simulink model "ranwalk_kalman"  (Simulink 5.0)
settings: Solver=ode45  StartTime=0.0  StopTime=100.0  RelTol=1e-3
values from neighbouring files (symbols this model uses):
  H = [1 0 1 1 1 1 1 1 1 1 1 1 ... (56 elements, 2x28)]    [cmigits28_model_01.mat]    (also in covanal.m = zeros(1,28))
  P0 = covupdate(P1,K,H)    [casimple.m]    (also in cmigits28_model_01.mat = [100 0 0 0 0 0 0 0 0 0 0 0 ... (784 elements, 28x28)])
  Phi = expm(F)    [casimple.m]    (also in covanal.m = eye(28))
  Q = [100 0 0 0 0 0 0 0 0 0 0 0 ... (784 elements, 28x28)]    [cmigits28_model_01.mat]    (also in covanal.m = eye(28))
  R = Re + h    (= 6378441.8)    [A-init.m]    (also in Ainit.m; cmigits28_model_01.mat = [50  0; 0  50]; covanal.m = zeros(1,1); covariance_analysis.m = meas_noise_growth_factor*R)
  x0 = [lat,lon,Vn,Ve,0,0,0,-R,0]'    [Ainit.m]
undefined symbols (not defined in the file or in its folder): rss_ratio, trace, ud_inv
libraries: simulink x4
settings Model: Creator=mcarroll  LastModifiedBy=mcarroll  ExtModeAutoUpdateStatusClock=off  SaveFormat=StructureWithTime

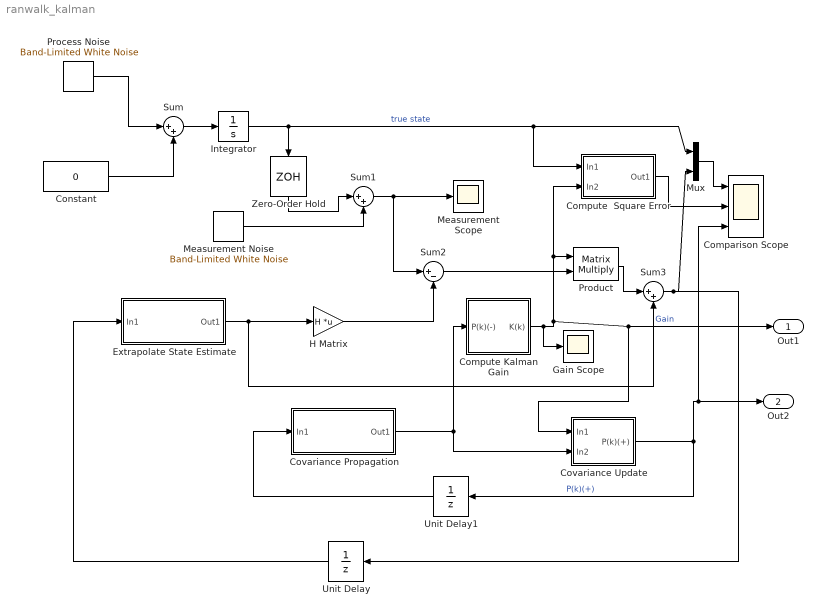
== system ranwalk_kalman ==
  Comparison Scope : Scope  NumInputPorts=3
      settings: TimeRange=100  YMin=1.5~-5~-5  YMax=6.5~5~5  SaveName=ScopeData12
  Compute Kalman Gain : Subsystem
  Compute  Square Error : Subsystem
  Constant : Constant  Value=0
  Covariance Propagation : Subsystem
  Covariance Update : Subsystem
  Extrapolate State Estimate : Subsystem
  Gain Scope : Scope
  H Matrix : Gain  Gain=H  Multiplication=Matrix(K*u)  SaturateOnIntegerOverflow=on
  Integrator : Integrator  InitialCondition=5+randn
  Measurement Noise : simulink/Sources/Band-Limited White Noise  Cov=[0.01]  Ts=0.1  seed=[23341]
  Measurement Scope : Scope
  Mux : Mux  Inputs=2
  Process Noise : simulink/Sources/Band-Limited White Noise  Cov=[10]  Ts=0.1  seed=[23341]
  Product : Product  Multiplication=Matrix(*)  SaturateOnIntegerOverflow=on
  Sum : Sum  Inputs=|++  SaturateOnIntegerOverflow=on
  Sum1 : Sum  Inputs=|++  SaturateOnIntegerOverflow=on
  Sum2 : Sum  Inputs=|+-  SaturateOnIntegerOverflow=on
  Sum3 : Sum  Inputs=|++  SaturateOnIntegerOverflow=on
  Unit Delay : UnitDelay  Orientation=left  X0=x0
  Unit Delay1 : UnitDelay  Orientation=left  X0=P0
  Zero-Order Hold : ZeroOrderHold  Orientation=down
  Out1 : Outport
  Out2 : Outport  Port=2
  wires:
  Sum/1 -> Integrator/1
  Process Noise/1 -> Sum/1
  Constant/1 -> Sum/2
  Integrator/1 -> Zero-Order Hold/1, Mux/1, Compute  Square Error/1(In1)  "true state"
  Measurement Noise/1 -> Sum1/2
  Sum1/1 -> Measurement Scope/1, Sum2/1
  Extrapolate State Estimate/1(Out1) -> H Matrix/1, Sum3/2
  H Matrix/1 -> Sum2/2
  Sum3/1 -> Unit Delay/1, Mux/2
  Unit Delay/1 -> Extrapolate State Estimate/1(In1)
  Zero-Order Hold/1 -> Sum1/1
  Unit Delay1/1 -> Covariance Propagation/1(In1)
  Covariance Propagation/1(Out1) -> Compute Kalman Gain/1(P(k)(-)), Covariance Update/2(In2)
  Compute Kalman Gain/1(K(k)) -> Covariance Update/1(In1), Out1/1, Product/1, Compute  Square Error/2(In2), Gain Scope/1  "Gain"
  Covariance Update/1(P(k)(+)) -> Unit Delay1/1, Out2/1, Comparison Scope/3  "P(k)(+)"
  Product/1 -> Sum3/1
  Sum2/1 -> Product/2
  Mux/1 -> Comparison Scope/1
  Compute  Square Error/1(Out1) -> Comparison Scope/2

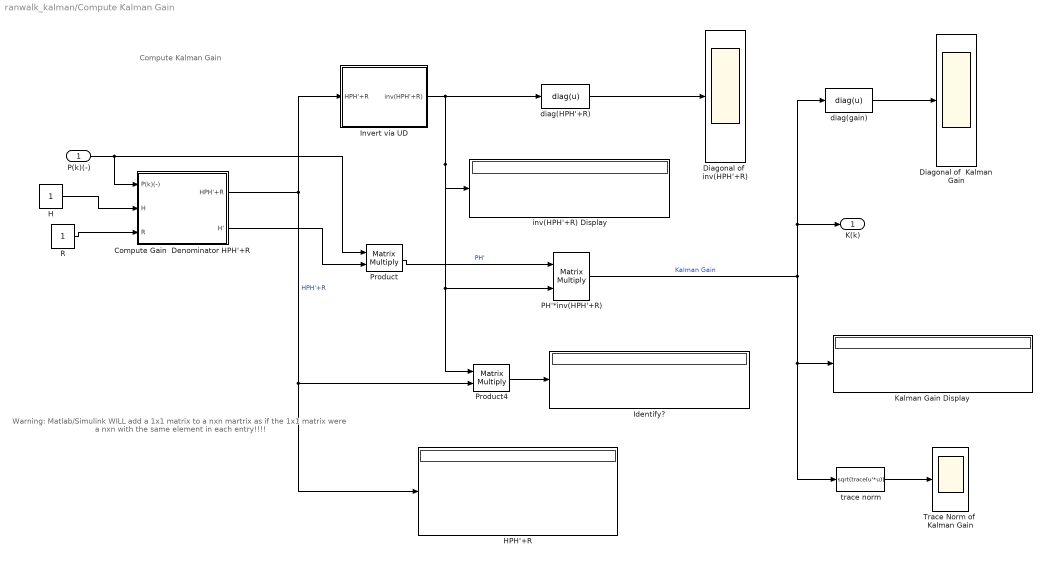
== system ranwalk_kalman/Compute Kalman Gain ==
  note: Compute Kalman Gain
  note: Warning:
      | Matlab/Simulink
      | WILL add a 1x1 matrix to
      | a nxn martrix as if the
      | 1x1 matrix were a
      | nxn with the same element
      | in each entry!!!!
  P(k)(-) : Inport  ShowAdditionalParam=on
  Compute Gain  Denominator HPH'+R : Subsystem
  Diagonal of  Kalman Gain : Scope
      settings: TimeRange=10  YMin=0  YMax=0.8  SaveName=ScopeData7
  Diagonal of  inv(HPH'+R) : Scope
      settings: TimeRange=100  YMin=0.0006  YMax=0.002  SaveName=ScopeData8
  H : Constant
  HPH'+R : Display
  Identify? : Display
  Invert via UD : Subsystem
  Kalman Gain Display : Display
  PH'*inv(HPH'+R) : Product  Multiplication=Matrix(*)  SaturateOnIntegerOverflow=on  InputSameDT=on
  Product : Product  Multiplication=Matrix(*)  SaturateOnIntegerOverflow=on
  Product4 : Product  Multiplication=Matrix(*)  SaturateOnIntegerOverflow=on  InputSameDT=on
  R : Constant
  Trace Norm of  Kalman Gain : Scope
      settings: TimeRange=10  YMin=0.5  YMax=0.62  SaveName=ScopeData11
  diag(HPH'+R) : MATLABFcn  MATLABFcn=diag(u)
  diag(gain) : MATLABFcn  MATLABFcn=diag(u)  Output1D=off
  inv(HPH'+R) Display : Display
  trace norm : MATLABFcn  MATLABFcn=sqrt(trace(u'*u))  Output1D=off
  K(k) : Outport
  wires:
  Compute Gain  Denominator HPH'+R/1(HPH'+R) -> Invert via UD/1(HPH'+R), HPH'+R/1, Product4/2  "HPH'+R"
  R/1 -> Compute Gain  Denominator HPH'+R/3(R)
  diag(HPH'+R)/1 -> Diagonal of  inv(HPH'+R)/1
  Invert via UD/1(inv(HPH'+R)) -> diag(HPH'+R)/1, inv(HPH'+R) Display/1, PH'*inv(HPH'+R)/2, Product4/1
  Compute Gain  Denominator HPH'+R/2(H') -> Product/2
  Product/1 -> PH'*inv(HPH'+R)/1  "PH'"
  diag(gain)/1 -> Diagonal of  Kalman Gain/1
  trace norm/1 -> Trace Norm of  Kalman Gain/1
  Product4/1 -> Identify?/1
  H/1 -> Compute Gain  Denominator HPH'+R/2(H)
  P(k)(-)/1 -> Compute Gain  Denominator HPH'+R/1(P(k)(-)), Product/1
  PH'*inv(HPH'+R)/1 -> K(k)/1, diag(gain)/1, Kalman Gain Display/1, trace norm/1  "Kalman Gain"

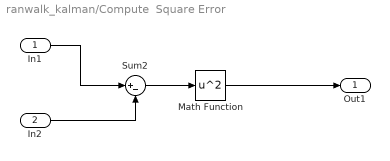
== system ranwalk_kalman/Compute  Square Error ==
  In1 : Inport
  In2 : Inport  Port=2
  Math Function : Math  Operator=square
  Sum2 : Sum  Inputs=|+-  SaturateOnIntegerOverflow=on
  Out1 : Outport
  wires:
  In1/1 -> Sum2/1
  In2/1 -> Sum2/2
  Sum2/1 -> Math Function/1
  Math Function/1 -> Out1/1

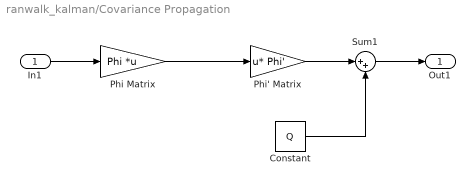
== system ranwalk_kalman/Covariance Propagation ==
  In1 : Inport
  Constant : Constant  Value=Q
  Phi Matrix : Gain  Gain=Phi  Multiplication=Matrix(K*u)  SaturateOnIntegerOverflow=on
  Phi' Matrix : Gain  Gain=Phi'  Multiplication=Matrix(u*K)  SaturateOnIntegerOverflow=on
  Sum1 : Sum  Inputs=|++  SaturateOnIntegerOverflow=on
  Out1 : Outport
  wires:
  In1/1 -> Phi Matrix/1
  Phi Matrix/1 -> Phi' Matrix/1
  Phi' Matrix/1 -> Sum1/1
  Constant/1 -> Sum1/2
  Sum1/1 -> Out1/1

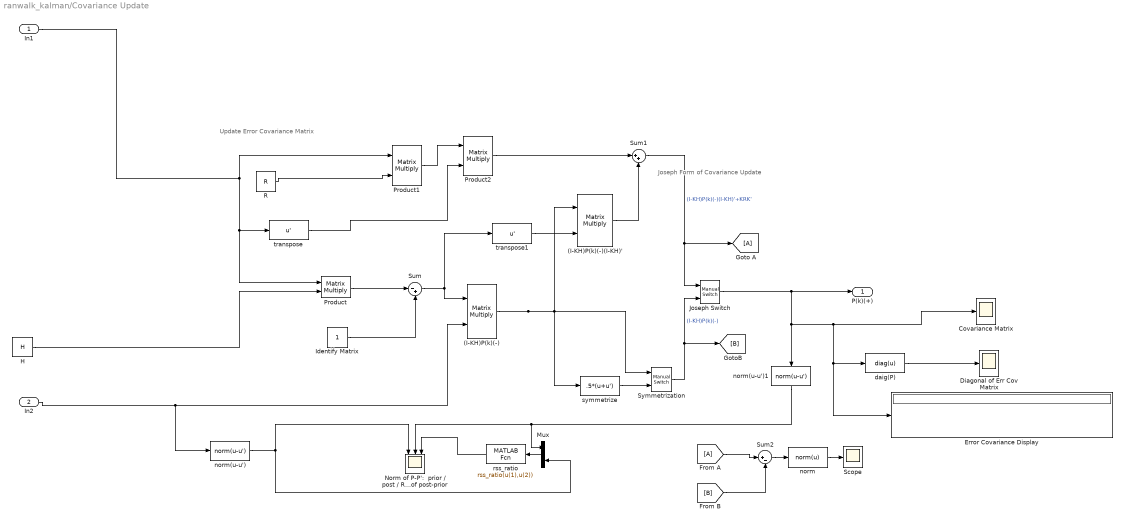
== system ranwalk_kalman/Covariance Update ==
  note: Update Error Covariance Matrix
  note: Joseph Form
      | of Covariance
      | Update
  In1 : Inport
  In2 : Inport  Port=2
  (I-KH)P(k)(-) : Product  Multiplication=Matrix(*)  SaturateOnIntegerOverflow=on  InputSameDT=on
  (I-KH)P(k)(-)(I-KH)' : Product  Multiplication=Matrix(*)  SaturateOnIntegerOverflow=on  InputSameDT=on
  Covariance Matrix : Scope
      settings: TimeRange=10  YMin=-60  YMax=80  SaveName=ScopeData2
  Diagonal of Err Cov Matrix : Scope
      settings: YMin=0  YMax=5000  SaveName=ScopeData3
  Error Covariance Display : Display
  H : Constant  Value=H  VectorParams1D=off
  Identify Matrix : Constant  VectorParams1D=off
  Joseph Switch : simulink/Signal Routing/Manual Switch  sw=1  action=0
  Mux : Mux  Orientation=left  Inputs=2
  Norm of P-P':  prior / post / RSS ratio of post-prior : Scope  NumInputPorts=3
      settings: Orientation=down  TimeRange=10  YMin=0~0~0  YMax=40~2~0.05  SaveName=ScopeData4
  Product : Product  Multiplication=Matrix(*)  SaturateOnIntegerOverflow=on  InputSameDT=on
  Product1 : Product  Multiplication=Matrix(*)  SaturateOnIntegerOverflow=on  InputSameDT=on
  Product2 : Product  Multiplication=Matrix(*)  ShowAdditionalParam=on  SaturateOnIntegerOverflow=on  InputSameDT=on
  R : Constant  Value=R  VectorParams1D=off
  Scope : Scope
      settings: SaveName=ScopeData5
  Sum : Sum  Inputs=|-+  SaturateOnIntegerOverflow=on  InputSameDT=on
  Sum1 : Sum  Inputs=|++  SaturateOnIntegerOverflow=on  InputSameDT=on
  Sum2 : Sum  Inputs=|+-  SaturateOnIntegerOverflow=on  InputSameDT=on
  Symmetrization : simulink/Signal Routing/Manual Switch  sw=1  action=0
  daig(P) : MATLABFcn  MATLABFcn=diag(u)
  norm : MATLABFcn  MATLABFcn=norm(u)  Output1D=off
  norm(u-u') : MATLABFcn  MATLABFcn=norm(u-u')  Output1D=off
  norm(u-u')1 : MATLABFcn  Orientation=down  MATLABFcn=norm(u-u')  Output1D=off
  rss_ratio : MATLABFcn  Orientation=left  MATLABFcn=rss_ratio(u(1),u(2))  OutputSignalType=real
  symmetrize : MATLABFcn  MATLABFcn=.5*(u+u')  Output1D=off
  transpose : MATLABFcn  MATLABFcn=u'  Output1D=off
  transpose1 : MATLABFcn  MATLABFcn=u'  Output1D=off
  P(k)(+) : Outport
  wires:
  H/1 -> Product/2
  In1/1 -> Product/1, transpose/1, Product1/1
  In2/1 -> (I-KH)P(k)(-)/2, norm(u-u')/1
  Identify Matrix/1 -> Sum/2
  Product/1 -> Sum/1
  Sum/1 -> (I-KH)P(k)(-)/1, transpose1/1
  R/1 -> Product1/2
  transpose/1 -> Product2/2
  (I-KH)P(k)(-)/1 -> (I-KH)P(k)(-)(I-KH)'/1, Symmetrization/1, symmetrize/1
  transpose1/1 -> (I-KH)P(k)(-)(I-KH)'/2
  (I-KH)P(k)(-)(I-KH)'/1 -> Sum1/2
  Product2/1 -> Sum1/1
  symmetrize/1 -> Symmetrization/2
  Symmetrization/1 -> Joseph Switch/2, [B]  "(I-KH)P(k)(-)"
  Joseph Switch/1 -> P(k)(+)/1, norm(u-u')1/1, daig(P)/1, Error Covariance Display/1, Covariance Matrix/1
  Sum1/1 -> Joseph Switch/1, [A]  "(I-KH)P(k)(-)(I-KH)'+KRK'"
  norm(u-u')/1 -> Norm of P-P':  prior / post / RSS ratio of post-prior/1, Mux/2
  norm(u-u')1/1 -> Norm of P-P':  prior / post / RSS ratio of post-prior/2, Mux/1
  rss_ratio/1 -> Norm of P-P':  prior / post / RSS ratio of post-prior/3
  Mux/1 -> rss_ratio/1
  [B] -> Sum2/2
  [A] -> Sum2/1
  Sum2/1 -> norm/1
  norm/1 -> Scope/1
  daig(P)/1 -> Diagonal of Err Cov Matrix/1
  Product1/1 -> Product2/1

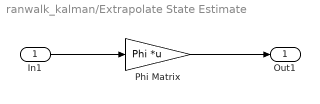
== system ranwalk_kalman/Extrapolate State Estimate ==
  In1 : Inport
  Phi Matrix : Gain  Gain=Phi  Multiplication=Matrix(K*u)  SaturateOnIntegerOverflow=on
  Out1 : Outport
  wires:
  In1/1 -> Phi Matrix/1
  Phi Matrix/1 -> Out1/1

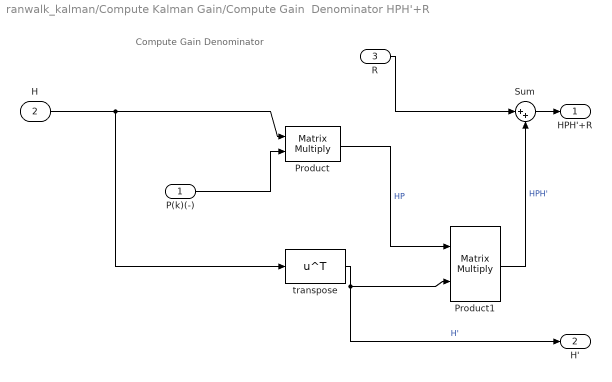
== system ranwalk_kalman/Compute Kalman Gain/Compute Gain  Denominator HPH'+R ==
  note: Compute Gain Denominator
  P(k)(-) : Inport
  H : Inport  Port=2
  R : Inport  Port=3
  Product : Product  Multiplication=Matrix(*)  SaturateOnIntegerOverflow=on  InputSameDT=on
  Product1 : Product  Multiplication=Matrix(*)  SaturateOnIntegerOverflow=on  InputSameDT=on
  Sum : Sum  Inputs=|++  SaturateOnIntegerOverflow=on  InputSameDT=on
  transpose : Math  Operator=transpose
  HPH'+R : Outport
  H' : Outport  Port=2
  wires:
  transpose/1 -> H'/1, Product1/2  "H'"
  Product1/1 -> Sum/2  "HPH'"
  Product/1 -> Product1/1  "HP"
  H/1 -> Product/1, transpose/1
  R/1 -> Sum/1
  Sum/1 -> HPH'+R/1
  P(k)(-)/1 -> Product/2

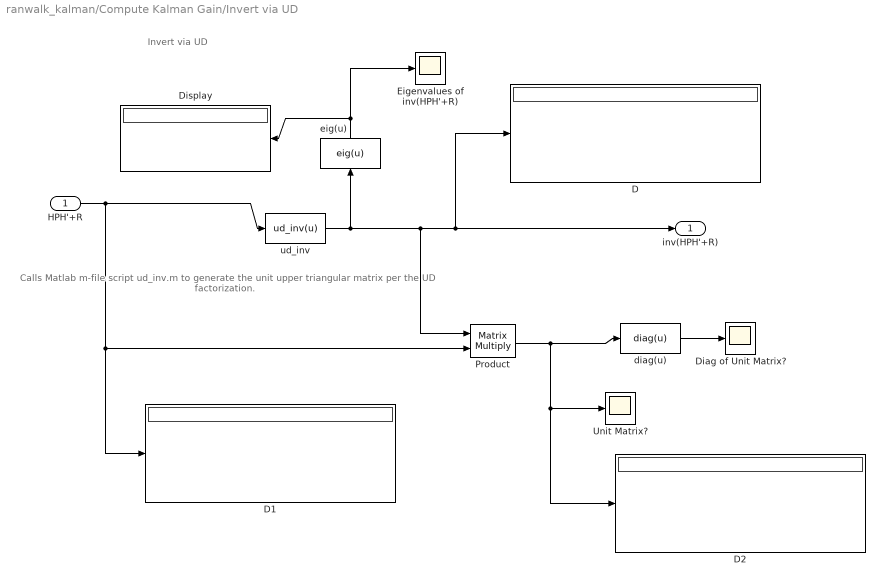
== system ranwalk_kalman/Compute Kalman Gain/Invert via UD ==
  note: Calls Matlab m-file script ud_inv.m
      | to generate the unit upper triangular
      | matrix per the UD factorization.
  note: Invert via UD
  HPH'+R : Inport
  D : Display
  D1 : Display
  D2 : Display
  Diag of Unit Matrix? : Scope
      settings: YMin=0.99  YMax=1.03  SaveName=ScopeData10
  Display : Display
  Eigenvalues of inv(HPH'+R) : Scope
      settings: SaveName=ScopeData6
  Product : Product  Multiplication=Matrix(*)  SaturateOnIntegerOverflow=on  InputSameDT=on
  Unit Matrix? : Scope
      settings: SaveName=ScopeData9
  diag(u) : MATLABFcn  MATLABFcn=diag(u)  Output1D=off
  eig(u) : MATLABFcn  Orientation=up  MATLABFcn=eig(u)  Output1D=off
  ud_inv : MATLABFcn  MATLABFcn=ud_inv(u)  Output1D=off
  inv(HPH'+R) : Outport
  wires:
  HPH'+R/1 -> ud_inv/1, D1/1, Product/2
  ud_inv/1 -> eig(u)/1, inv(HPH'+R)/1, D/1, Product/1
  eig(u)/1 -> Eigenvalues of inv(HPH'+R)/1, Display/1
  Product/1 -> diag(u)/1, Unit Matrix?/1, D2/1
  diag(u)/1 -> Diag of Unit Matrix?/1
